simulink model "IEEE_BUS_68_Baseline"  (R2025a)
settings: Solver=ode23tb  StartTime=0.0  StopTime=150  FixedStep=Ts  MaxStep=0.0001  RelTol=1e-3
PreLoadFcn:
  | PSSMODEL=1;
  | LPSS=0;
  | WAPSS=0;
  | WAPSS2=0;
  | Ts=50e-5;
InitFcn:
  | PSSMODEL=1;
  | LPSS=0;
  | WAPSS=0;
  | WAPSS2=0;
  | Ts=50e-5;
  | 
  | % Required data to 68 Bus benchmark
  | % clear
  | % clc
  | % Definition for the columns
  | % system base =100 MVA
  | 
  | %% Line data Format (line)
  | % All values are given on the same system base MVA
  | % 1: From bus
  | % 2: To bus
  | % 3: Resistance (pu)
  | % 4: Reactance  (pu)
  | % 5: Charge     (pu)
  | % 6: Transformer Tap Amplitute
  | % 7: base MVA
  | % 8: Nomonal Voltage (KV)
  | 
  | %1   2    3        4       5       6        7      8
  | line=[...
  | 1	54	0	     0.0181	  0	      1.025     100    13.8
  | 2	58	0	     0.025	  0	      1.070     100    13.8
  | 3	62	0	     0.02	  0	      1.070     100    13.8
  | 4	19	0.0007	 0.0142	  0	      1.070     100    13.8
  | 5	20	0.0009	 0.018	  0	      1.009     100    13.8
  | 6	22	0	     0.0143	  0	      1.025     100    13.8
  | 7	23	0.0005	 0.0272	  0	      0         100    13.8
  | 8	25	0.0006	 0.0232	  0	      1.025     100    13.8
  | 9	29	0.0008	 0.0156   0	      1.025     100    13.8
  | 10	31	0	     0.026	  0	      1.04      100    13.8
  | 11	32	0	     0.013	  0	      1.04      100    13.8
  | 12	36	0	     0.0075	  0	      1.04      100    13.8
  | 13	17	0	     0.0033	  0	      1.04      100    13.8
  | 14	41	0	     0.0015	  0	      1         100    13.8
  | 15	42	0	     0.0015	  0	      1         100    13.8
  | 16	18	0	     0.003	  0	      1         100    13.8
  | 17	36	0.0005	 0.0045	  0.32	  0         100    138
  | 17	43	0.0005	 0.0276	  0	      0         100    138
  | 18	42	0.004	 0.06	  2.25    0         100    138
  | 18	49	0.0076	 0.1141	  1.16    0	        100    138
  | 18	50	0.0012	 0.0288	  2.06	  0         100    138
  | 20	19	0.0007	 0.0138	  0       1.06	    100    138
  | 19	68	0.0016	 0.0195	  0.304	  0         100    138
  | 21	22	0.0008	 0.014	  0.2565  0	        100    138
  | 21	68	0.0008	 0.0135	  0.2548  0	        100    138
  | 22	23	0.0006	 0.0096	  0.1846  0	        100    138
  | 23	24	0.0022	 0.035	  0.361	  0         100    138
  | 24	68	0.0003	 0.0059	  0.068	  0         100    138
  | 25	26	0.0032	 0.0323	  0.531	  0         100    138
  | 25	54	0.007	 0.0086	  0.146	  0         100    138
  | 26	27	0.0014	 0.0147	  0.2396  0	        100    138
  | 26	28	0.0043	 0.0474	  0.7802  0	        100    138
  | 26	29	0.0057	 0.0625	  1.029	  0         100    138
  | 27	37	0.0013	 0.0173	  0.3216  0	        100    138
  | 27	53	0.032	 0.32	  0.41	  0         100    138
  | ... (+206 lines)
undefined symbols (not defined in the file or in its folder): D1, Delta
libraries: spsRMSLib x73, spsThreePhaseVIMeasurementLib x69, spsLoadFlowBusLib x69, spsThreePhasePISectionLineLib x64, spsThreePhaseParallelRLCLoadLib x35, spsGenericPowerSystemStabilizerLib x32, spsThreePhaseSeriesRLCLoadLib x21, spsThreePhaseTransformerTwoWindingsLib x21, spsSynchronousMachinepuStandardLib x19, spsExcitationSystemLib x16, spsMultiBandPowerSystemStabilizerLib x16, spsSteamTurbineandGovernorLib x16
(part 2 of 7)

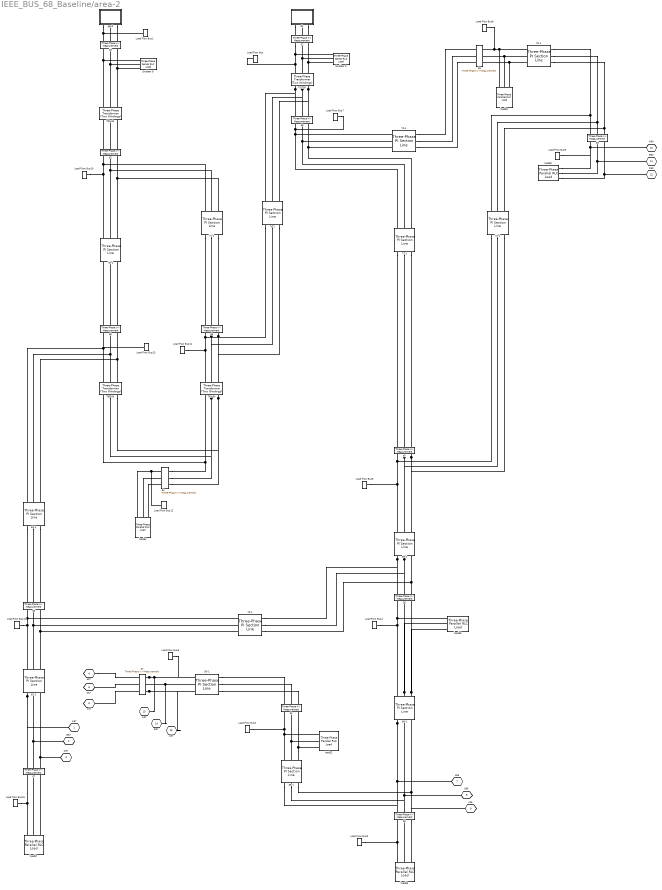
== system IEEE_BUS_68_Baseline/area-2 ==
  02 : spsThreePhaseVIMeasurementLib/Three-Phase V-I Measurement  VoltageMeasurement=phase-to-phase  SetLabelV=on  LabelV=Vabc_02  Vpu=off  VpuLL=on  CurrentMeasurement=no  SetLabelI=off  LabelI=Iabc  Ipu=off  Pbase=100e6  Vbase=13.8e3  OutputType=Complex  PhasorSimulation=off  PSBequivalent=0
  03 : spsThreePhaseVIMeasurementLib/Three-Phase V-I Measurement  VoltageMeasurement=phase-to-phase  SetLabelV=on  LabelV=Vabc_03  Vpu=off  VpuLL=on  CurrentMeasurement=no  SetLabelI=off  LabelI=Iabc  Ipu=off  Pbase=100e6  Vbase=13.8e3  OutputType=Complex  PhasorSimulation=off  PSBequivalent=0
  37 : spsThreePhaseVIMeasurementLib/Three-Phase V-I Measurement  VoltageMeasurement=phase-to-phase  SetLabelV=on  LabelV=Vabc_37  Vpu=off  VpuLL=on  CurrentMeasurement=no  SetLabelI=off  LabelI=Iabc  Ipu=off  Pbase=100e6  Vbase=Bus(37,2)*1e3  OutputType=Complex  PhasorSimulation=off  PSBequivalent=0
  50-1 : spsThreePhasePISectionLineLib/Three-Phase PI Section Line  LConnTagsString=a|b|c  RConnTagsString=A|B|C  Length=1  Frequency=60  Resistances=[line(50,3) 3*line(50,3)]  Inductances=[line(50,4) 3*line(50,4)]  Capacitances=[line(50,5) line(50,5)/3]
  52 : spsThreePhaseVIMeasurementLib/Three-Phase V-I Measurement  VoltageMeasurement=phase-to-phase  SetLabelV=on  LabelV=Vabc_52  Vpu=off  VpuLL=on  CurrentMeasurement=no  SetLabelI=off  LabelI=Iabc  Ipu=off  Pbase=100e6  Vbase=Bus(52,2)*1e3  OutputType=Complex  PhasorSimulation=off  PSBequivalent=0
  55 : spsThreePhaseVIMeasurementLib/Three-Phase V-I Measurement  VoltageMeasurement=phase-to-phase  SetLabelV=on  LabelV=Vabc_55  Vpu=off  VpuLL=on  CurrentMeasurement=no  SetLabelI=off  LabelI=Iabc  Ipu=off  Pbase=100e6  Vbase=Bus(55,2)*1e3  OutputType=Complex  PhasorSimulation=off  PSBequivalent=0
  56 : spsThreePhaseVIMeasurementLib/Three-Phase V-I Measurement  VoltageMeasurement=phase-to-phase  SetLabelV=on  LabelV=Vabc_56  Vpu=off  VpuLL=on  CurrentMeasurement=no  SetLabelI=off  LabelI=Iabc  Ipu=off  Pbase=100e6  Vbase=Bus(56,2)*1e3  OutputType=Complex  PhasorSimulation=off  PSBequivalent=0
  57 : spsThreePhaseVIMeasurementLib/Three-Phase V-I Measurement  VoltageMeasurement=phase-to-phase  SetLabelV=on  LabelV=Vabc_57  Vpu=off  VpuLL=on  CurrentMeasurement=no  SetLabelI=off  LabelI=Iabc  Ipu=off  Pbase=100e6  Vbase=Bus(57,2)*1e3  OutputType=Complex  PhasorSimulation=off  PSBequivalent=0
  58 : spsThreePhaseVIMeasurementLib/Three-Phase V-I Measurement  VoltageMeasurement=phase-to-phase  SetLabelV=on  LabelV=Vabc_58  Vpu=off  VpuLL=on  CurrentMeasurement=no  SetLabelI=off  LabelI=Iabc  Ipu=off  Pbase=100e6  Vbase=Bus(58,2)*1e3  OutputType=Complex  PhasorSimulation=off  PSBequivalent=0
  59 : spsThreePhaseVIMeasurementLib/Three-Phase V-I Measurement  VoltageMeasurement=phase-to-phase  SetLabelV=on  LabelV=Vabc_59  Vpu=off  VpuLL=on  CurrentMeasurement=no  SetLabelI=off  LabelI=Iabc  Ipu=off  Pbase=100e6  Vbase=Bus(59,2)*1e3  OutputType=Complex  PhasorSimulation=off  PSBequivalent=0
  60 : spsThreePhaseVIMeasurementLib/Three-Phase V-I Measurement  VoltageMeasurement=phase-to-phase  SetLabelV=on  LabelV=Vabc_60  Vpu=off  VpuLL=on  CurrentMeasurement=no  SetLabelI=off  LabelI=Iabc  Ipu=off  Pbase=100e6  Vbase=Bus(60,2)*1e3  OutputType=Complex  PhasorSimulation=off  PSBequivalent=0
  62 : spsThreePhaseVIMeasurementLib/Three-Phase V-I Measurement  VoltageMeasurement=phase-to-phase  SetLabelV=on  LabelV=Vabc_62  Vpu=off  VpuLL=on  CurrentMeasurement=no  SetLabelI=off  LabelI=Iabc  Ipu=off  Pbase=100e6  Vbase=Bus(62,2)*1e3  OutputType=Complex  PhasorSimulation=off  PSBequivalent=0
  63 : spsThreePhaseVIMeasurementLib/Three-Phase V-I Measurement  VoltageMeasurement=phase-to-phase  SetLabelV=on  LabelV=Vabc_63  Vpu=off  VpuLL=on  CurrentMeasurement=no  SetLabelI=off  LabelI=Iabc  Ipu=off  Pbase=100e6  Vbase=Bus(63,2)*1e3  OutputType=Complex  PhasorSimulation=off  PSBequivalent=0
  64 : spsThreePhaseVIMeasurementLib/Three-Phase V-I Measurement  VoltageMeasurement=phase-to-phase  SetLabelV=on  LabelV=Vabc_64  Vpu=off  VpuLL=on  CurrentMeasurement=no  SetLabelI=off  LabelI=Iabc  Ipu=off  Pbase=100e6  Vbase=Bus(64,2)*1e3  OutputType=Complex  PhasorSimulation=off  PSBequivalent=0
  65 : spsThreePhaseVIMeasurementLib/Three-Phase V-I Measurement  VoltageMeasurement=phase-to-phase  SetLabelV=on  LabelV=Vabc_65  Vpu=off  VpuLL=on  CurrentMeasurement=no  SetLabelI=off  LabelI=Iabc  Ipu=off  Pbase=100e6  Vbase=Bus(65,2)*1e3  OutputType=Complex  PhasorSimulation=off  PSBequivalent=0
  65-1 : spsThreePhasePISectionLineLib/Three-Phase PI Section Line  LConnTagsString=a|b|c  RConnTagsString=A|B|C  Length=1  Frequency=60  Resistances=[line(65,3) 3*line(65,3)]  Inductances=[line(65,4) 3*line(65,4)]  Capacitances=[line(65,5) line(65,5)/3]
  66 : spsThreePhaseVIMeasurementLib/Three-Phase V-I Measurement  VoltageMeasurement=phase-to-phase  SetLabelV=on  LabelV=Vabc_66  Vpu=off  VpuLL=on  CurrentMeasurement=no  SetLabelI=off  LabelI=Iabc  Ipu=off  Pbase=100e6  Vbase=Bus(66,2)*1e3  OutputType=Complex  PhasorSimulation=off  PSBequivalent=0
  67 : spsThreePhaseVIMeasurementLib/Three-Phase V-I Measurement  VoltageMeasurement=phase-to-phase  SetLabelV=on  LabelV=Vabc_67  Vpu=off  VpuLL=on  CurrentMeasurement=no  SetLabelI=off  LabelI=Iabc  Ipu=off  Pbase=100e6  Vbase=Bus(67,2)*1e3  OutputType=Complex  PhasorSimulation=off  PSBequivalent=0
  68-1 : spsThreePhasePISectionLineLib/Three-Phase PI Section Line  LConnTagsString=a|b|c  RConnTagsString=A|B|C  Length=1  Frequency=60  Resistances=[line(68,3) 3*line(68,3)]  Inductances=[line(68,4) 3*line(68,4)]  Capacitances=[line(68,5) line(68,5)/3]
  69-1 : spsThreePhasePISectionLineLib/Three-Phase PI Section Line  LConnTagsString=a|b|c  RConnTagsString=A|B|C  Length=1  Frequency=60  Resistances=[line(69,3) 3*line(69,3)]  Inductances=[line(69,4) 3*line(69,4)]  Capacitances=[line(69,5) line(69,5)/3]
  70-1 : spsThreePhasePISectionLineLib/Three-Phase PI Section Line  LConnTagsString=a|b|c  RConnTagsString=A|B|C  Length=1  Frequency=60  Resistances=[line(70,3) 3*line(70,3)]  Inductances=[line(70,4) 3*line(70,4)]  Capacitances=[line(70,5) line(70,5)/3]
  71-1 : spsThreePhasePISectionLineLib/Three-Phase PI Section Line  LConnTagsString=a|b|c  RConnTagsString=A|B|C  Length=1  Frequency=60  Resistances=[line(71,3) 3*line(71,3)]  Inductances=[line(71,4) 3*line(71,4)]  Capacitances=[line(71,5) line(71,5)/3]
  72-1 : spsThreePhasePISectionLineLib/Three-Phase PI Section Line  LConnTagsString=a|b|c  RConnTagsString=A|B|C  Length=1  Frequency=60  Resistances=[line(72,3) 3*line(72,3)]  Inductances=[line(72,4) 3*line(72,4)]  Capacitances=[line(72,5) line(72,5)/3]
  73-1 : spsThreePhasePISectionLineLib/Three-Phase PI Section Line  LConnTagsString=a|b|c  RConnTagsString=A|B|C  Length=1  Frequency=60  Resistances=[line(73,3) 3*line(73,3)]  Inductances=[line(73,4) 3*line(73,4)]  Capacitances=[line(73,5) line(73,5)/3]
  74-1 : spsThreePhasePISectionLineLib/Three-Phase PI Section Line  LConnTagsString=a|b|c  RConnTagsString=A|B|C  Length=1  Frequency=60  Resistances=[line(74,3) 3*line(74,3)]  Inductances=[line(74,4) 3*line(74,4)]  Capacitances=[line(74,5) line(74,5)/3]
  75-1 : spsThreePhasePISectionLineLib/Three-Phase PI Section Line  LConnTagsString=a|b|c  RConnTagsString=A|B|C  Length=1  Frequency=60  Resistances=[line(75,3) 3*line(75,3)]  Inductances=[line(75,4) 3*line(75,4)]  Capacitances=[line(75,5) line(75,5)/3]
  77-1 : spsThreePhasePISectionLineLib/Three-Phase PI Section Line  LConnTagsString=a|b|c  RConnTagsString=A|B|C  Length=1  Frequency=60  Resistances=[line(77,3) 3*line(77,3)]  Inductances=[line(77,4) 3*line(77,4)]  Capacitances=[line(77,5) line(77,5)/3]
  78-1 : spsThreePhasePISectionLineLib/Three-Phase PI Section Line  LConnTagsString=a|b|c  RConnTagsString=A|B|C  Length=1  Frequency=60  Resistances=[line(78,3) 3*line(78,3)]  Inductances=[line(78,4) 3*line(78,4)]  Capacitances=[line(78,5) line(78,5)/3]
  81-1 : spsThreePhasePISectionLineLib/Three-Phase PI Section Line  LConnTagsString=a|b|c  RConnTagsString=A|B|C  Length=1  Frequency=60  Resistances=[line(81,3) 3*line(81,3)]  Inductances=[line(81,4) 3*line(81,4)]  Capacitances=[line(81,5) line(81,5)/3]
  81-2 : spsThreePhasePISectionLineLib/Three-Phase PI Section Line  LConnTagsString=a|b|c  RConnTagsString=A|B|C  Length=1  Frequency=60  Resistances=[line(81,3) 3*line(81,3)]  Inductances=[line(81,4) 3*line(81,4)]  Capacitances=[line(81,5) line(81,5)/3]
  G2 : Subsystem
  Load Flow Bus : spsLoadFlowBusLib/Load Flow Bus  LConnTagsString=a  Phases=single  Connectors=on one side  ID=BUS_02  Vbase=13.8e3  Vref=0.98  Vangle=0  VLF=0.98  VLFb=1  VLFc=1  angleLF=-3.815  angleLFb=0  angleLFc=0
  Load Flow Bus1 : spsLoadFlowBusLib/Load Flow Bus  LConnTagsString=a  Phases=single  Connectors=on one side  ID=BUS_03  Vbase=13.8e3  Vref=0.983  Vangle=0  VLF=0.983  VLFb=1  VLFc=1  angleLF=2.903  angleLFb=0  angleLFc=0
  Load Flow Bus10 : spsLoadFlowBusLib/Load Flow Bus  LConnTagsString=a  Phases=single  Connectors=on one side  ID=BUS_62  Vbase=138e3  Vref=1  Vangle=0  VLF=0.9822  VLFb=1  VLFc=1  angleLF=29.01  angleLFb=0  angleLFc=0
  Load Flow Bus11 : spsLoadFlowBusLib/Load Flow Bus  LConnTagsString=a  Phases=single  Connectors=on one side  ID=BUS_63  Vbase=138e3  Vref=1  Vangle=0  VLF=0.9798  VLFb=1  VLFc=1  angleLF=28.04  angleLFb=0  angleLFc=0
  Load Flow Bus12 : spsLoadFlowBusLib/Load Flow Bus  LConnTagsString=a  Phases=single  Connectors=on one side  ID=BUS_64  Vbase=138e3  Vref=1  Vangle=0  VLF=0.971  VLFb=1  VLFc=1  angleLF=28.2  angleLFb=0  angleLFc=0
  Load Flow Bus13 : spsLoadFlowBusLib/Load Flow Bus  LConnTagsString=a  Phases=single  Connectors=on one side  ID=BUS_65  Vbase=138e3  Vref=1  Vangle=0  VLF=0.9825  VLFb=1  VLFc=1  angleLF=28.32  angleLFb=0  angleLFc=0
  Load Flow Bus14 : spsLoadFlowBusLib/Load Flow Bus  LConnTagsString=a  Phases=single  Connectors=on one side  ID=BUS_66  Vbase=138e3  Vref=1  Vangle=0  VLF=0.9879  VLFb=1  VLFc=1  angleLF=26.8  angleLFb=0  angleLFc=0
  Load Flow Bus15 : spsLoadFlowBusLib/Load Flow Bus  LConnTagsString=a  Phases=single  Connectors=on one side  ID=BUS_67  Vbase=138e3  Vref=1  Vangle=0  VLF=0.9975  VLFb=1  VLFc=1  angleLF=26.93  angleLFb=0  angleLFc=0
  Load Flow Bus2 : spsLoadFlowBusLib/Load Flow Bus  LConnTagsString=a  Phases=single  Connectors=on one side  ID=BUS_52  Vbase=138e3  Vref=1  Vangle=0  VLF=1.004  VLFb=1  VLFc=1  angleLF=24.49  angleLFb=0  angleLFc=0
  Load Flow Bus3 : spsLoadFlowBusLib/Load Flow Bus  LConnTagsString=a  Phases=single  Connectors=on one side  ID=BUS_55  Vbase=138e3  Vref=1  Vangle=0  VLF=0.9927  VLFb=1  VLFc=1  angleLF=22.46  angleLFb=0  angleLFc=0
  Load Flow Bus4 : spsLoadFlowBusLib/Load Flow Bus  LConnTagsString=a  Phases=single  Connectors=on one side  ID=BUS_56  Vbase=138e3  Vref=1  Vangle=0  VLF=0.9814  VLFb=1  VLFc=1  angleLF=24.68  angleLFb=0  angleLFc=0
  Load Flow Bus5 : spsLoadFlowBusLib/Load Flow Bus  LConnTagsString=a  Phases=single  Connectors=on one side  ID=BUS_37  Vbase=138e3  Vref=1  Vangle=0  VLF=1.011  VLFb=1  VLFc=1  angleLF=25.73  angleLFb=0  angleLFc=0
  Load Flow Bus6 : spsLoadFlowBusLib/Load Flow Bus  LConnTagsString=a  Phases=single  Connectors=on one side  ID=BUS_57  Vbase=138e3  Vref=1  Vangle=0  VLF=0.9776  VLFb=1  VLFc=1  angleLF=25.41  angleLFb=0  angleLFc=0
  Load Flow Bus7 : spsLoadFlowBusLib/Load Flow Bus  LConnTagsString=a  Phases=single  Connectors=on one side  ID=BUS_58  Vbase=138e3  Vref=1  Vangle=0  VLF=0.9787  VLFb=1  VLFc=1  angleLF=26.13  angleLFb=0  angleLFc=0
  Load Flow Bus8 : spsLoadFlowBusLib/Load Flow Bus  LConnTagsString=a  Phases=single  Connectors=on one side  ID=BUS_59  Vbase=138e3  Vref=1  Vangle=0  VLF=0.9693  VLFb=1  VLFc=1  angleLF=23.58  angleLFb=0  angleLFc=0
  Load Flow Bus9 : spsLoadFlowBusLib/Load Flow Bus  LConnTagsString=a  Phases=single  Connectors=on one side  ID=BUS_60  Vbase=138e3  Vref=1  Vangle=0  VLF=0.9693  VLFb=1  VLFc=1  angleLF=22.93  angleLFb=0  angleLFc=0
  Snubber 8 : spsThreePhaseSeriesRLCLoadLib/Three-Phase Series RLC Load  LConnTagsString=A|B|C  Configuration=Y (grounded)  NominalVoltage=13.8e3  Vabc=[1e3 1e3 1e3]  Vabcp=[1e3 1e3 1e3]  NominalFrequency=60  UnbalancedPower=off  ActivePower=1000000  InductivePower=0  CapacitivePower=10000000  Pabc=[10e3 9e3 11e3]  QLabc=[100 90 110]  QCabc=[100 90 110]  Pabcp=[10e3 9e3 11e3]  QLabcp=[100 90 110]  QCabcp=[100 90 110]  Measurements=None  LoadType=constant Z
  Snubber 9 : spsThreePhaseSeriesRLCLoadLib/Three-Phase Series RLC Load  LConnTagsString=A|B|C  Configuration=Y (grounded)  NominalVoltage=13.8e3  Vabc=[1e3 1e3 1e3]  Vabcp=[1e3 1e3 1e3]  NominalFrequency=60  UnbalancedPower=off  ActivePower=1000000  InductivePower=0  CapacitivePower=10000000  Pabc=[10e3 9e3 11e3]  QLabc=[100 90 110]  QCabc=[100 90 110]  Pabcp=[10e3 9e3 11e3]  QLabcp=[100 90 110]  QCabcp=[100 90 110]  Measurements=None  LoadType=constant Z
  T02-58 : spsThreePhaseTransformerTwoWindingsLib/Three-Phase Transformer (Two Windings)  Winding1Connection=Delta (D1)  Winding2Connection=Yg  CoreType=Three single-phase transformers  SetSaturation=off  Hysteresis=off  DataFile='hysteresis'  SetInitialFlux=off  Measurements=None  UNITS=pu  NominalPower=[ 100e6 , 60 ]  Winding1=[ 13.8e3 , 0.0002 , 0 ]  Winding2=[ 138e3 , 0 .0002, 0.0125]  Rm=500  Lm=500  L0=0.5  Saturation=[ 0,0 ; 0.0024,1.2 ; 1.0,1.52 ]  InitialFluxes=[ 0.8 , -0.8 , 0.7 ]  BreakLoop=off  DiscreteSolver=Trapezoidal robust  DataType=off  TransfoNumber=1
  T03-62 : spsThreePhaseTransformerTwoWindingsLib/Three-Phase Transformer (Two Windings)  Winding1Connection=Delta (D1)  Winding2Connection=Yg  CoreType=Three single-phase transformers  SetSaturation=off  Hysteresis=off  DataFile='hysteresis'  SetInitialFlux=off  Measurements=None  UNITS=pu  NominalPower=[ 100e6 , 60 ]  Winding1=[ 13.8e3 , 0.000 , 0 ]  Winding2=[ 138e3 , 0.000, 0.0101]  Rm=500  Lm=500  L0=0.5  Saturation=[ 0,0 ; 0.0024,1.2 ; 1.0,1.52 ]  InitialFluxes=[ 0.8 , -0.8 , 0.7 ]  BreakLoop=off  DiscreteSolver=Trapezoidal robust  DataType=off  TransfoNumber=1
  T63-64 : spsThreePhaseTransformerTwoWindingsLib/Three-Phase Transformer (Two Windings)  Winding1Connection=Y  Winding2Connection=Y  CoreType=Three single-phase transformers  SetSaturation=off  Hysteresis=off  DataFile='hysteresis'  SetInitialFlux=off  Measurements=None  UNITS=pu  NominalPower=[ 100e6 , 60 ]  Winding1=[ 138e3 , 0.00152, 0 ]  Winding2=[ 138e3 , 0.00152 , 0.022]  Rm=500  Lm=500  L0=0.5  Saturation=[ 0,0 ; 0.0024,1.2 ; 1.0,1.52 ]  InitialFluxes=[ 0.8 , -0.8 , 0.7 ]  BreakLoop=off  DiscreteSolver=Trapezoidal robust  DataType=off  TransfoNumber=1
  T65-64 : spsThreePhaseTransformerTwoWindingsLib/Three-Phase Transformer (Two Windings)  Winding1Connection=Y  Winding2Connection=Y  CoreType=Three single-phase transformers  SetSaturation=off  Hysteresis=off  DataFile='hysteresis'  SetInitialFlux=off  Measurements=None  UNITS=pu  NominalPower=[ 100e6 , 60 ]  Winding1=[ 138e3 , 0.00152, 0 ]  Winding2=[ 138e3 , 0.00152 , 0.022]  Rm=500  Lm=500  L0=0.5  Saturation=[ 0,0 ; 0.0024,1.2 ; 1.0,1.52 ]  InitialFluxes=[ 0.8 , -0.8 , 0.7 ]  BreakLoop=off  DiscreteSolver=Trapezoidal robust  DataType=off  TransfoNumber=1
  gen3 : Subsystem
  load52 : spsThreePhaseParallelRLCLoadLib/Three-Phase Parallel RLC Load  LConnTagsString=A|B|C  Configuration=Y (grounded)  NominalVoltage=(138000)*1.00427  Vabc=[1e3 1e3 1e3]  Vabcp=[1e3 1e3 1e3]  NominalFrequency=60  UnbalancedPower=off  ActivePower=2000000  InductivePower=460000  CapacitivePower=0  Pabc=[10e3 9e3 11e3]  QLabc=[100 90 110]  QCabc=[100 90 110]  Pabcp=[10e3 9e3 11e3]  QLabcp=[100 90 110]  QCabcp=[100 90 110]  Measurements=None  LoadType=constant PQ
  load55 : spsThreePhaseParallelRLCLoadLib/Three-Phase Parallel RLC Load  LConnTagsString=A|B|C  Configuration=Y (grounded)  NominalVoltage=(138000)*0.992749  Vabc=[1e3 1e3 1e3]  Vabcp=[1e3 1e3 1e3]  NominalFrequency=60  UnbalancedPower=off  ActivePower=680000000  InductivePower=157000000  CapacitivePower=0  Pabc=[10e3 9e3 11e3]  QLabc=[100 90 110]  QCabc=[100 90 110]  Pabcp=[10e3 9e3 11e3]  QLabcp=[100 90 110]  QCabcp=[100 90 110]  Measurements=None  LoadType=constant PQ
  load56 : spsThreePhaseParallelRLCLoadLib/Three-Phase Parallel RLC Load  LConnTagsString=A|B|C  Configuration=Y (grounded)  NominalVoltage=(138000)*0.981401  Vabc=[1e3 1e3 1e3]  Vabcp=[1e3 1e3 1e3]  NominalFrequency=60  UnbalancedPower=off  ActivePower=200000000  InductivePower=74000000  CapacitivePower=0  Pabc=[10e3 9e3 11e3]  QLabc=[100 90 110]  QCabc=[100 90 110]  Pabcp=[10e3 9e3 11e3]  QLabcp=[100 90 110]  QCabcp=[100 90 110]  Measurements=None  LoadType=constant PQ
  load59 : spsThreePhaseParallelRLCLoadLib/Three-Phase Parallel RLC Load  LConnTagsString=A|B|C  Configuration=Y (grounded)  NominalVoltage=(138000)*0.969335  Vabc=[1e3 1e3 1e3]  Vabcp=[1e3 1e3 1e3]  NominalFrequency=60  UnbalancedPower=off  ActivePower=234000000  InductivePower=84000000  CapacitivePower=0  Pabc=[10e3 9e3 11e3]  QLabc=[100 90 110]  QCabc=[100 90 110]  Pabcp=[10e3 9e3 11e3]  QLabcp=[100 90 110]  QCabcp=[100 90 110]  Measurements=None  LoadType=constant PQ
  load60 : spsThreePhaseParallelRLCLoadLib/Three-Phase Parallel RLC Load  LConnTagsString=A|B|C  Configuration=Y (grounded)  NominalVoltage=(138000)*0.969257  Vabc=[1e3 1e3 1e3]  Vabcp=[1e3 1e3 1e3]  NominalFrequency=60  UnbalancedPower=off  ActivePower=209000000  InductivePower=71000000  CapacitivePower=0  Pabc=[10e3 9e3 11e3]  QLabc=[100 90 110]  QCabc=[100 90 110]  Pabcp=[10e3 9e3 11e3]  QLabcp=[100 90 110]  QCabcp=[100 90 110]  Measurements=None  LoadType=constant PQ
  load64 : spsThreePhaseParallelRLCLoadLib/Three-Phase Parallel RLC Load  LConnTagsString=A|B|C  Configuration=Y (grounded)  NominalVoltage=(138000)*0.971036  Vabc=[1e3 1e3 1e3]  Vabcp=[1e3 1e3 1e3]  NominalFrequency=60  UnbalancedPower=off  ActivePower=9000000  InductivePower=88000000  CapacitivePower=0  Pabc=[10e3 9e3 11e3]  QLabc=[100 90 110]  QCabc=[100 90 110]  Pabcp=[10e3 9e3 11e3]  QLabcp=[100 90 110]  QCabcp=[100 90 110]  Measurements=None  LoadType=constant PQ
  load67 : spsThreePhaseParallelRLCLoadLib/Three-Phase Parallel RLC Load  LConnTagsString=A|B|C  Configuration=Y (grounded)  NominalVoltage=(138000)*0.997526  Vabc=[1e3 1e3 1e3]  Vabcp=[1e3 1e3 1e3]  NominalFrequency=60  UnbalancedPower=off  ActivePower=118000000  InductivePower=27000000  CapacitivePower=0  Pabc=[10e3 9e3 11e3]  QLabc=[100 90 110]  QCabc=[100 90 110]  Pabcp=[10e3 9e3 11e3]  QLabcp=[100 90 110]  QCabcp=[100 90 110]  Measurements=None  LoadType=constant PQ
  A67 : PMIOPort  Tag=PMCPort  Side=Right
  B67 : PMIOPort  Tag=PMCPort  Port=2  Side=Right
  C67 : PMIOPort  Tag=PMCPort  Port=3  Side=Right
  a37 : PMIOPort  Tag=PMCPort  Port=4  Side=Right
  c37 : PMIOPort  Tag=PMCPort  Port=5  Side=Right
  b37 : PMIOPort  Tag=PMCPort  Port=6  Side=Right
  a55 : PMIOPort  Tag=PMCPort  Port=7  Side=Right
  b55 : PMIOPort  Tag=PMCPort  Port=8  Side=Right
  c55 : PMIOPort  Tag=PMCPort  Port=9  Side=Right
  A60 : PMIOPort  Tag=PMCPort  Port=10  Side=Right
  B60 : PMIOPort  Tag=PMCPort  Port=11  Side=Right
  C60 : PMIOPort  Tag=PMCPort  Port=12  Side=Right
  A37 : PMIOPort  Tag=PMCPort  Port=13  Side=Right
  B37 : PMIOPort  Tag=PMCPort  Port=14  Side=Right
  C37 : PMIOPort  Tag=PMCPort  Port=15  Side=Right
  connections:
  gen3/LConn2 -- 03/RConn2
  62/RConn3 -- T03-62/RConn3
  T03-62/LConn1 -- 03/LConn1 -- Snubber 8/LConn1
  T03-62/LConn2 -- 03/LConn2 -- Snubber 8/LConn2
  62/RConn2 -- T03-62/RConn2
  62/RConn1 -- T03-62/RConn1
  gen3/LConn3 -- 03/RConn3
  gen3/LConn1 -- Load Flow Bus1/LConn1 -- 03/RConn1
  T03-62/LConn3 -- Snubber 8/LConn3 -- 03/LConn3
  78-1/RConn1 -- Load Flow Bus10/LConn1 -- 77-1/RConn1 -- 62/LConn1
  78-1/RConn2 -- 77-1/RConn2 -- 62/LConn2
  78-1/RConn3 -- 77-1/RConn3 -- 62/LConn3
  65/RConn1 -- 78-1/LConn1
  65/RConn2 -- 78-1/LConn2
  65/RConn3 -- 78-1/LConn3
  77-1/LConn1 -- 63/RConn1
  77-1/LConn2 -- 63/RConn2
  77-1/LConn3 -- 63/RConn3
  T63-64/LConn1 -- Load Flow Bus11/LConn1 -- 63/LConn1 -- 74-1/RConn1
  63/LConn2 -- T63-64/LConn2 -- 74-1/RConn2
  63/LConn3 -- T63-64/LConn3 -- 74-1/RConn3
  64/RConn1 -- T63-64/RConn1 -- T65-64/RConn1
  T63-64/RConn2 -- 64/RConn2 -- T65-64/RConn2
  T63-64/RConn3 -- 64/RConn3 -- T65-64/RConn3
  T65-64/LConn1 -- Load Flow Bus13/LConn1 -- 65/LConn1 -- 81-1/RConn1
  T65-64/LConn2 -- 81-1/RConn2 -- 65/LConn2
  T65-64/LConn3 -- 81-1/RConn3 -- 65/LConn3
  load64/LConn1 -- Load Flow Bus12/LConn1 -- 64/LConn1
  load64/LConn2 -- 64/LConn2
  load64/LConn3 -- 64/LConn3
  81-1/LConn1 -- 66/RConn1
  81-1/LConn2 -- 66/RConn2
  81-1/LConn3 -- 66/RConn3
  81-2/RConn1 -- Load Flow Bus14/LConn1 -- 66/LConn1 -- 70-1/RConn1
  81-2/RConn2 -- 66/LConn2 -- 70-1/RConn2
  81-2/RConn3 -- 66/LConn3 -- 70-1/RConn3
  81-2/LConn1 -- 67/RConn1 -- A67/RConn1
  67/RConn2 -- 81-2/LConn2 -- B67/RConn1
  C67/RConn1 -- 67/RConn3 -- 81-2/LConn3
  G2/LConn1 -- 02/RConn1
  G2/LConn2 -- 02/RConn2
  G2/LConn3 -- 02/RConn3
  02/LConn1 -- Snubber 9/LConn1 -- Load Flow Bus/LConn1 -- T02-58/LConn1
  T02-58/LConn2 -- 02/LConn2 -- Snubber 9/LConn2
  T02-58/LConn3 -- Snubber 9/LConn3 -- 02/LConn3
  T02-58/RConn1 -- 58/RConn1 -- 74-1/LConn1
  T02-58/RConn2 -- 58/RConn2 -- 74-1/LConn2
  T02-58/RConn3 -- 58/RConn3 -- 74-1/LConn3
  73-1/RConn1 -- 71-1/RConn1 -- Load Flow Bus7/LConn1 -- 58/LConn1
  71-1/RConn2 -- 73-1/RConn2 -- 58/LConn2
  71-1/RConn3 -- 73-1/RConn3 -- 58/LConn3
  71-1/LConn1 -- 57/RConn1
  71-1/LConn2 -- 57/RConn2
  71-1/LConn3 -- 57/RConn3
  73-1/LConn1 -- 59/RConn1
  73-1/LConn2 -- 59/RConn2
  73-1/LConn3 -- 59/RConn3
  75-1/RConn1 -- load59/LConn1 -- Load Flow Bus8/LConn1 -- 59/LConn1
  75-1/RConn2 -- load59/LConn2 -- 59/LConn2
  75-1/RConn3 -- load59/LConn3 -- 59/LConn3
  75-1/LConn1 -- 60/RConn1 -- 72-1/LConn1
  75-1/LConn2 -- 60/RConn2 -- 72-1/LConn2
  75-1/LConn3 -- 60/RConn3 -- 72-1/LConn3
  A60/RConn1 -- load60/LConn1 -- Load Flow Bus9/LConn1 -- 60/LConn1
  load60/LConn2 -- 60/LConn2 -- B60/RConn1
  load60/LConn3 -- C60/RConn1 -- 60/LConn3
  69-1/RConn1 -- 57/LConn1 -- 72-1/RConn1 -- Load Flow Bus6/LConn1
  57/LConn2 -- 69-1/RConn2 -- 72-1/RConn2
  57/LConn3 -- 69-1/RConn3 -- 72-1/RConn3
  69-1/LConn1 -- 56/RConn1 -- 70-1/LConn1
  69-1/LConn2 -- 56/RConn2 -- 70-1/LConn2
  56/RConn3 -- 70-1/LConn3 -- 69-1/LConn3
  68-1/RConn1 -- Load Flow Bus4/LConn1 -- load56/LConn1 -- 56/LConn1
  68-1/RConn2 -- load56/LConn2 -- 56/LConn2
  68-1/RConn3 -- load56/LConn3 -- 56/LConn3
  68-1/LConn1 -- 55/RConn1 -- 65-1/LConn1 -- a55/RConn1
  b55/RConn1 -- 55/RConn2 -- 65-1/LConn2 -- 68-1/LConn2
  65-1/LConn3 -- 68-1/LConn3 -- 55/RConn3 -- c55/RConn1
  load67/LConn1 -- Load Flow Bus15/LConn1 -- 67/LConn1
  load67/LConn2 -- 67/LConn2
  load67/LConn3 -- 67/LConn3
  65-1/RConn1 -- 52/LConn1 -- Load Flow Bus2/LConn1 -- load52/LConn1
  65-1/RConn2 -- load52/LConn2 -- 52/LConn2
  65-1/RConn3 -- load52/LConn3 -- 52/LConn3
  Load Flow Bus3/LConn1 -- 55/LConn1 -- load55/LConn1
  a37/RConn1 -- 37/RConn1
  37/RConn2 -- b37/RConn1
  37/RConn3 -- c37/RConn1
  37/LConn1 -- Load Flow Bus5/LConn1 -- 50-1/RConn1 -- A37/RConn1
  50-1/RConn2 -- B37/RConn1 -- 37/LConn2
  37/LConn3 -- 50-1/RConn3 -- C37/RConn1
  50-1/LConn1 -- 52/RConn1
  50-1/LConn2 -- 52/RConn2
  50-1/LConn3 -- 52/RConn3
  load55/LConn2 -- 55/LConn2
  load55/LConn3 -- 55/LConn3

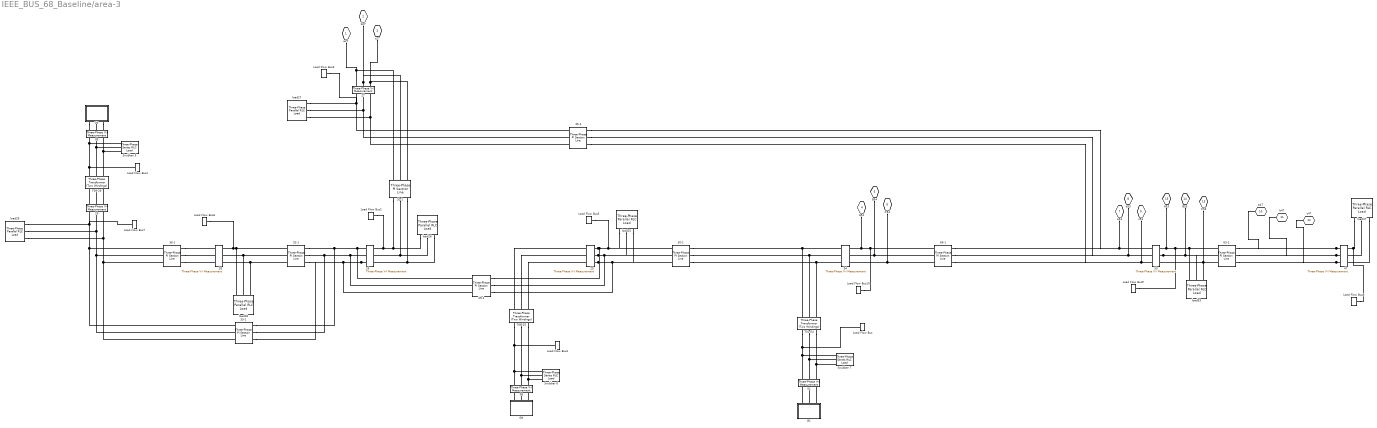
== system IEEE_BUS_68_Baseline/area-3 ==
  01 : spsThreePhaseVIMeasurementLib/Three-Phase V-I Measurement  VoltageMeasurement=phase-to-phase  SetLabelV=on  LabelV=Vabc_01  Vpu=off  VpuLL=on  CurrentMeasurement=no  SetLabelI=off  LabelI=Iabc  Ipu=off  Pbase=100e6  Vbase=13.8e3  OutputType=Complex  PhasorSimulation=off  PSBequivalent=0
  08 : spsThreePhaseVIMeasurementLib/Three-Phase V-I Measurement  VoltageMeasurement=phase-to-phase  SetLabelV=on  LabelV=Vabc_08  Vpu=off  VpuLL=on  CurrentMeasurement=no  SetLabelI=off  LabelI=Iabc  Ipu=off  Pbase=100e6  Vbase=13.8e3  OutputType=Complex  PhasorSimulation=off  PSBequivalent=0
  09 : spsThreePhaseVIMeasurementLib/Three-Phase V-I Measurement  VoltageMeasurement=phase-to-phase  SetLabelV=on  LabelV=Vabc_09  Vpu=off  VpuLL=on  CurrentMeasurement=no  SetLabelI=off  LabelI=Iabc  Ipu=off  Pbase=100e6  Vbase=13.8e3  OutputType=Complex  PhasorSimulation=off  PSBequivalent=0
  25 : spsThreePhaseVIMeasurementLib/Three-Phase V-I Measurement  VoltageMeasurement=phase-to-phase  SetLabelV=on  LabelV=Vabc_25  Vpu=off  VpuLL=on  CurrentMeasurement=no  SetLabelI=off  LabelI=Iabc  Ipu=off  Pbase=100e6  Vbase=Bus(25,2)*1e3  OutputType=Complex  PhasorSimulation=off  PSBequivalent=0
  26 : spsThreePhaseVIMeasurementLib/Three-Phase V-I Measurement  VoltageMeasurement=phase-to-phase  SetLabelV=on  LabelV=Vabc_26  Vpu=off  VpuLL=on  CurrentMeasurement=no  SetLabelI=off  LabelI=Iabc  Ipu=off  Pbase=100e6  Vbase=Bus(26,2)*1e3  OutputType=Complex  PhasorSimulation=off  PSBequivalent=0
  27 : spsThreePhaseVIMeasurementLib/Three-Phase V-I Measurement  VoltageMeasurement=phase-to-phase  SetLabelV=on  LabelV=Vabc_27  Vpu=off  VpuLL=on  CurrentMeasurement=no  SetLabelI=off  LabelI=Iabc  Ipu=off  Pbase=100e6  Vbase=Bus(27,2)*1e3  OutputType=Complex  PhasorSimulation=off  PSBequivalent=0
  28 : spsThreePhaseVIMeasurementLib/Three-Phase V-I Measurement  VoltageMeasurement=phase-to-phase  SetLabelV=on  LabelV=Vabc_28  Vpu=off  VpuLL=on  CurrentMeasurement=no  SetLabelI=off  LabelI=Iabc  Ipu=off  Pbase=100e6  Vbase=Bus(28,2)*1e3  OutputType=Complex  PhasorSimulation=off  PSBequivalent=0
  29 : spsThreePhaseVIMeasurementLib/Three-Phase V-I Measurement  VoltageMeasurement=phase-to-phase  SetLabelV=on  LabelV=Vabc_29  Vpu=off  VpuLL=on  CurrentMeasurement=no  SetLabelI=off  LabelI=Iabc  Ipu=off  Pbase=100e6  Vbase=Bus(29,2)*1e3  OutputType=Complex  PhasorSimulation=off  PSBequivalent=0
  29-1 : spsThreePhasePISectionLineLib/Three-Phase PI Section Line  LConnTagsString=a|b|c  RConnTagsString=A|B|C  Length=1  Frequency=60  Resistances=[line(29,3) 3*line(29,3)]  Inductances=[line(29,4) 3*line(29,4)]  Capacitances=[line(29,5) line(29,5)/3]
  30-1 : spsThreePhasePISectionLineLib/Three-Phase PI Section Line  LConnTagsString=a|b|c  RConnTagsString=A|B|C  Length=1  Frequency=60  Resistances=[line(30,3) 3*line(30,3)]  Inductances=[line(30,4) 3*line(30,4)]  Capacitances=[line(30,5) line(30,5)/3]
  31-1 : spsThreePhasePISectionLineLib/Three-Phase PI Section Line  LConnTagsString=a|b|c  RConnTagsString=A|B|C  Length=1  Frequency=60  Resistances=[line(31,3) 3*line(31,3)]  Inductances=[line(31,4) 3*line(31,4)]  Capacitances=[line(31,5) line(31,5)/3]
  32-1 : spsThreePhasePISectionLineLib/Three-Phase PI Section Line  LConnTagsString=a|b|c  RConnTagsString=A|B|C  Length=1  Frequency=60  Resistances=[line(32,3) 3*line(32,3)]  Inductances=[line(32,4) 3*line(32,4)]  Capacitances=[line(32,5) line(32,5)/3]
  33-1 : spsThreePhasePISectionLineLib/Three-Phase PI Section Line  LConnTagsString=a|b|c  RConnTagsString=A|B|C  Length=1  Frequency=60  Resistances=[line(33,3) 3*line(33,3)]  Inductances=[line(33,4) 3*line(33,4)]  Capacitances=[line(33,5) line(33,5)/3]
  35-1 : spsThreePhasePISectionLineLib/Three-Phase PI Section Line  LConnTagsString=a|b|c  RConnTagsString=A|B|C  Length=1  Frequency=60  Resistances=[line(35,3) 3*line(35,3)]  Inductances=[line(35,4) 3*line(35,4)]  Capacitances=[line(35,5) line(35,5)/3]
  36-1 : spsThreePhasePISectionLineLib/Three-Phase PI Section Line  LConnTagsString=a|b|c  RConnTagsString=A|B|C  Length=1  Frequency=60  Resistances=[line(36,3) 3*line(36,3)]  Inductances=[line(36,4) 3*line(36,4)]  Capacitances=[line(36,5) line(36,5)/3]
  47 : spsThreePhaseVIMeasurementLib/Three-Phase V-I Measurement  VoltageMeasurement=phase-to-phase  SetLabelV=on  LabelV=Vabc_47  Vpu=off  VpuLL=on  CurrentMeasurement=no  SetLabelI=off  LabelI=Iabc  Ipu=off  Pbase=100e6  Vbase=Bus(47,2)*1e3  OutputType=Complex  PhasorSimulation=off  PSBequivalent=0
  53 : spsThreePhaseVIMeasurementLib/Three-Phase V-I Measurement  VoltageMeasurement=phase-to-phase  SetLabelV=on  LabelV=Vabc_53  Vpu=off  VpuLL=on  CurrentMeasurement=no  SetLabelI=off  LabelI=Iabc  Ipu=off  Pbase=100e6  Vbase=Bus(53,2)*1e3  OutputType=Complex  PhasorSimulation=off  PSBequivalent=0
  54 : spsThreePhaseVIMeasurementLib/Three-Phase V-I Measurement  VoltageMeasurement=phase-to-phase  SetLabelV=on  LabelV=Vabc_54  Vpu=off  VpuLL=on  CurrentMeasurement=no  SetLabelI=off  LabelI=Iabc  Ipu=off  Pbase=100e6  Vbase=Bus(54,2)*1e3  OutputType=Complex  PhasorSimulation=off  PSBequivalent=0
  63-1 : spsThreePhasePISectionLineLib/Three-Phase PI Section Line  LConnTagsString=a|b|c  RConnTagsString=A|B|C  Length=1  Frequency=60  Resistances=[line(63,3) 3*line(63,3)]  Inductances=[line(63,4) 3*line(63,4)]  Capacitances=[line(63,5) line(63,5)/3]
  66-1 : spsThreePhasePISectionLineLib/Three-Phase PI Section Line  LConnTagsString=a|b|c  RConnTagsString=A|B|C  Length=1  Frequency=60  Resistances=[line(66,3) 3*line(66,3)]  Inductances=[line(66,4) 3*line(66,4)]  Capacitances=[line(66,5) line(66,5)/3]
  G1 : Subsystem
  G8 : Subsystem
  G9 : Subsystem
  Load Flow Bus : spsLoadFlowBusLib/Load Flow Bus  LConnTagsString=a  Phases=single  Connectors=on one side  ID=BUS_01  Vbase=13.8e3  Vref=1.045  Vangle=0  VLF=1.045  VLFb=1  VLFc=1  angleLF=-3.223  angleLFb=0  angleLFc=0
  Load Flow Bus1 : spsLoadFlowBusLib/Load Flow Bus  LConnTagsString=a  Phases=single  Connectors=on one side  ID=BUS_09  Vbase=13.8e3  Vref=1.025  Vangle=0  VLF=1.025  VLFb=1  VLFc=1  angleLF=3.208  angleLFb=0  angleLFc=0
  Load Flow Bus10 : spsLoadFlowBusLib/Load Flow Bus  LConnTagsString=a  Phases=single  Connectors=on one side  ID=BUS_54  Vbase=138e3  Vref=1  Vangle=0  VLF=1.016  VLFb=1  VLFc=1  angleLF=24.39  angleLFb=0  angleLFc=0
  Load Flow Bus2 : spsLoadFlowBusLib/Load Flow Bus  LConnTagsString=a  Phases=single  Connectors=on one side  ID=BUS_26  Vbase=138e3  Vref=1  Vangle=0  VLF=1.035  VLFb=1  VLFc=1  angleLF=25.02  angleLFb=0  angleLFc=0
  Load Flow Bus3 : spsLoadFlowBusLib/Load Flow Bus  LConnTagsString=a  Phases=single  Connectors=on one side  ID=BUS_27  Vbase=138e3  Vref=1  Vangle=0  VLF=1.025  VLFb=1  VLFc=1  angleLF=24.61  angleLFb=0  angleLFc=0
  Load Flow Bus4 : spsLoadFlowBusLib/Load Flow Bus  LConnTagsString=a  Phases=single  Connectors=on one side  ID=BUS_08  Vbase=13.8e3  Vref=1.03  Vangle=0  VLF=1.03  VLFb=1  VLFc=1  angleLF=2.567  angleLFb=0  angleLFc=0
  Load Flow Bus5 : spsLoadFlowBusLib/Load Flow Bus  LConnTagsString=a  Phases=single  Connectors=on one side  ID=BUS_25  Vbase=138e3  Vref=1  Vangle=0  VLF=1.031  VLFb=1  VLFc=1  angleLF=25.81  angleLFb=0  angleLFc=0
  Load Flow Bus6 : spsLoadFlowBusLib/Load Flow Bus  LConnTagsString=a  Phases=single  Connectors=on one side  ID=BUS_28  Vbase=138e3  Vref=1  Vangle=0  VLF=1.028  VLFb=1  VLFc=1  angleLF=25.71  angleLFb=0  angleLFc=0
  Load Flow Bus7 : spsLoadFlowBusLib/Load Flow Bus  LConnTagsString=a  Phases=single  Connectors=on one side  ID=BUS_29  Vbase=138e3  Vref=1  Vangle=0  VLF=1.019  VLFb=1  VLFc=1  angleLF=26.38  angleLFb=0  angleLFc=0
  Load Flow Bus8 : spsLoadFlowBusLib/Load Flow Bus  LConnTagsString=a  Phases=single  Connectors=on one side  ID=BUS_47  Vbase=138e3  Vref=1  Vangle=0  VLF=1.013  VLFb=1  VLFc=1  angleLF=17.53  angleLFb=0  angleLFc=0
  Load Flow Bus9 : spsLoadFlowBusLib/Load Flow Bus  LConnTagsString=a  Phases=single  Connectors=on one side  ID=BUS_53  Vbase=138e3  Vref=1  Vangle=0  VLF=1.006  VLFb=1  VLFc=1  angleLF=18.11  angleLFb=0  angleLFc=0
  Snubber 5 : spsThreePhaseSeriesRLCLoadLib/Three-Phase Series RLC Load  LConnTagsString=A|B|C  Configuration=Y (grounded)  NominalVoltage=13.8e3  Vabc=[1e3 1e3 1e3]  Vabcp=[1e3 1e3 1e3]  NominalFrequency=60  UnbalancedPower=off  ActivePower=1000000  InductivePower=0  CapacitivePower=10000000  Pabc=[10e3 9e3 11e3]  QLabc=[100 90 110]  QCabc=[100 90 110]  Pabcp=[10e3 9e3 11e3]  QLabcp=[100 90 110]  QCabcp=[100 90 110]  Measurements=None  LoadType=constant Z
  Snubber 6 : spsThreePhaseSeriesRLCLoadLib/Three-Phase Series RLC Load  LConnTagsString=A|B|C  Configuration=Y (grounded)  NominalVoltage=13.8e3  Vabc=[1e3 1e3 1e3]  Vabcp=[1e3 1e3 1e3]  NominalFrequency=60  UnbalancedPower=off  ActivePower=1000000  InductivePower=0  CapacitivePower=10000000  Pabc=[10e3 9e3 11e3]  QLabc=[100 90 110]  QCabc=[100 90 110]  Pabcp=[10e3 9e3 11e3]  QLabcp=[100 90 110]  QCabcp=[100 90 110]  Measurements=None  LoadType=constant Z
  Snubber 7 : spsThreePhaseSeriesRLCLoadLib/Three-Phase Series RLC Load  LConnTagsString=A|B|C  Configuration=Y (grounded)  NominalVoltage=13.8e3  Vabc=[1e3 1e3 1e3]  Vabcp=[1e3 1e3 1e3]  NominalFrequency=60  UnbalancedPower=off  ActivePower=1000000  InductivePower=0  CapacitivePower=10000000  Pabc=[10e3 9e3 11e3]  QLabc=[100 90 110]  QCabc=[100 90 110]  Pabcp=[10e3 9e3 11e3]  QLabcp=[100 90 110]  QCabcp=[100 90 110]  Measurements=None  LoadType=constant Z
  T01-54 : spsThreePhaseTransformerTwoWindingsLib/Three-Phase Transformer (Two Windings)  Winding1Connection=Delta (D1)  Winding2Connection=Yg  CoreType=Three single-phase transformers  SetSaturation=off  Hysteresis=off  DataFile='hysteresis'  SetInitialFlux=off  Measurements=None  UNITS=pu  NominalPower=[ 100e6 , 60 ]  Winding1=[ 13.8e3 , 0.0002 , 0 ]  Winding2=[ 138e3 , 0.0002, 0.0181]  Rm=500  Lm=500  L0=0.5  Saturation=[ 0,0 ; 0.0024,1.2 ; 1.0,1.52 ]  InitialFluxes=[ 0.8 , -0.8 , 0.7 ]  BreakLoop=off  DiscreteSolver=Trapezoidal robust  DataType=off  TransfoNumber=1
  T08-25 : spsThreePhaseTransformerTwoWindingsLib/Three-Phase Transformer (Two Windings)  Winding1Connection=Delta (D1)  Winding2Connection=Yg  CoreType=Three single-phase transformers  SetSaturation=off  Hysteresis=off  DataFile='hysteresis'  SetInitialFlux=off  Measurements=None  UNITS=pu  NominalPower=[ 100e6 , 60 ]  Winding1=[ 13.8e3 , 0.0003 , 0 ]  Winding2=[ 138e3 , 0.0003, 0.0232]  Rm=500  Lm=500  L0=0.5  Saturation=[ 0,0 ; 0.0024,1.2 ; 1.0,1.52 ]  InitialFluxes=[ 0.8 , -0.8 , 0.7 ]  BreakLoop=off  DiscreteSolver=Trapezoidal robust  DataType=off  TransfoNumber=1
  T09-29 : spsThreePhaseTransformerTwoWindingsLib/Three-Phase Transformer (Two Windings)  Winding1Connection=Delta (D1)  Winding2Connection=Yg  CoreType=Three single-phase transformers  SetSaturation=off  Hysteresis=off  DataFile='hysteresis'  SetInitialFlux=off  Measurements=None  UNITS=pu  NominalPower=[ 100e6 , 60 ]  Winding1=[ 13.8e3 , 0.0004 , 0 ]  Winding2=[ 138e3 , 0.0004 , 0.0156]  Rm=500  Lm=500  L0=0.5  Saturation=[ 0,0 ; 0.0024,1.2 ; 1.0,1.52 ]  InitialFluxes=[ 0.8 , -0.8 , 0.7 ]  BreakLoop=off  DiscreteSolver=Trapezoidal robust  DataType=off  TransfoNumber=1
  load25 : spsThreePhaseParallelRLCLoadLib/Three-Phase Parallel RLC Load  LConnTagsString=A|B|C  Configuration=Y (grounded)  NominalVoltage=(138000)*1.03069  Vabc=[1e3 1e3 1e3]  Vabcp=[1e3 1e3 1e3]  NominalFrequency=60  UnbalancedPower=off  ActivePower=224000000  InductivePower=47000000  CapacitivePower=0  Pabc=[10e3 9e3 11e3]  QLabc=[100 90 110]  QCabc=[100 90 110]  Pabcp=[10e3 9e3 11e3]  QLabcp=[100 90 110]  QCabcp=[100 90 110]  Measurements=None  LoadType=constant PQ
  load26 : spsThreePhaseParallelRLCLoadLib/Three-Phase Parallel RLC Load  LConnTagsString=A|B|C  Configuration=Y (grounded)  NominalVoltage=(138000)*1.03482  Vabc=[1e3 1e3 1e3]  Vabcp=[1e3 1e3 1e3]  NominalFrequency=60  UnbalancedPower=off  ActivePower=50000000  InductivePower=7000000  CapacitivePower=0  Pabc=[10e3 9e3 11e3]  QLabc=[100 90 110]  QCabc=[100 90 110]  Pabcp=[10e3 9e3 11e3]  QLabcp=[100 90 110]  QCabcp=[100 90 110]  Measurements=None  LoadType=constant PQ
  load27 : spsThreePhaseParallelRLCLoadLib/Three-Phase Parallel RLC Load  LConnTagsString=A|B|C  Configuration=Y (grounded)  NominalVoltage=(138000)*1.02463  Vabc=[1e3 1e3 1e3]  Vabcp=[1e3 1e3 1e3]  NominalFrequency=60  UnbalancedPower=off  ActivePower=130000000  InductivePower=20000000  CapacitivePower=0  Pabc=[10e3 9e3 11e3]  QLabc=[100 90 110]  QCabc=[100 90 110]  Pabcp=[10e3 9e3 11e3]  QLabcp=[100 90 110]  QCabcp=[100 90 110]  Measurements=None  LoadType=constant PQ
  load28 : spsThreePhaseParallelRLCLoadLib/Three-Phase Parallel RLC Load  LConnTagsString=A|B|C  Configuration=Y (grounded)  NominalVoltage=(138000)*1.0279  Vabc=[1e3 1e3 1e3]  Vabcp=[1e3 1e3 1e3]  NominalFrequency=60  UnbalancedPower=off  ActivePower=50000000  InductivePower=7000000  CapacitivePower=0  Pabc=[10e3 9e3 11e3]  QLabc=[100 90 110]  QCabc=[100 90 110]  Pabcp=[10e3 9e3 11e3]  QLabcp=[100 90 110]  QCabcp=[100 90 110]  Measurements=None  LoadType=constant PQ
  load29 : spsThreePhaseParallelRLCLoadLib/Three-Phase Parallel RLC Load  LConnTagsString=A|B|C  Configuration=Y (grounded)  NominalVoltage=(138000)*1.01949  Vabc=[1e3 1e3 1e3]  Vabcp=[1e3 1e3 1e3]  NominalFrequency=60  UnbalancedPower=off  ActivePower=680000000  InductivePower=106000000  CapacitivePower=0  Pabc=[10e3 9e3 11e3]  QLabc=[100 90 110]  QCabc=[100 90 110]  Pabcp=[10e3 9e3 11e3]  QLabcp=[100 90 110]  QCabcp=[100 90 110]  Measurements=None  LoadType=constant PQ
  load47 : spsThreePhaseParallelRLCLoadLib/Three-Phase Parallel RLC Load  LConnTagsString=A|B|C  Configuration=Y (grounded)  NominalVoltage=(138000)*1.01263  Vabc=[1e3 1e3 1e3]  Vabcp=[1e3 1e3 1e3]  NominalFrequency=60  UnbalancedPower=off  ActivePower=203000000  InductivePower=33000000  CapacitivePower=0  Pabc=[10e3 9e3 11e3]  QLabc=[100 90 110]  QCabc=[100 90 110]  Pabcp=[10e3 9e3 11e3]  QLabcp=[100 90 110]  QCabcp=[100 90 110]  Measurements=None  LoadType=constant PQ
  load53 : spsThreePhaseParallelRLCLoadLib/Three-Phase Parallel RLC Load  LConnTagsString=A|B|C  Configuration=Y (grounded)  NominalVoltage=(138000)*1.00612  Vabc=[1e3 1e3 1e3]  Vabcp=[1e3 1e3 1e3]  NominalFrequency=60  UnbalancedPower=off  ActivePower=253000000  InductivePower=119000000  CapacitivePower=0  Pabc=[10e3 9e3 11e3]  QLabc=[100 90 110]  QCabc=[100 90 110]  Pabcp=[10e3 9e3 11e3]  QLabcp=[100 90 110]  QCabcp=[100 90 110]  Measurements=None  LoadType=constant PQ
  a27 : PMIOPort  Tag=PMCPort  Side=Right
  b27 : PMIOPort  Tag=PMCPort  Port=2  Side=Right
  c27 : PMIOPort  Tag=PMCPort  Port=3  Side=Right
  A54 : PMIOPort  Tag=PMCPort  Port=4  Side=Right
  B54 : PMIOPort  Tag=PMCPort  Port=5  Side=Right
  C54 : PMIOPort  Tag=PMCPort  Port=6  Side=Right
  a53 : PMIOPort  Tag=PMCPort  Port=7  Side=Right
  b53 : PMIOPort  Tag=PMCPort  Port=8  Side=Right
  c53 : PMIOPort  Tag=PMCPort  Port=9  Side=Right
  a47 : PMIOPort  Tag=PMCPort  Port=10  Side=Right
  b47 : PMIOPort  Tag=PMCPort  Port=11  Side=Right
  c47 : PMIOPort  Tag=PMCPort  Port=12  Side=Right
  C53 : PMIOPort  Tag=PMCPort  Port=13  Side=Right
  B53 : PMIOPort  Tag=PMCPort  Port=14  Side=Right
  A53 : PMIOPort  Tag=PMCPort  Port=15  Side=Right
  connections:
  T09-29/LConn1 -- Snubber 5/LConn1 -- 09/LConn1 -- Load Flow Bus1/LConn1
  G9/LConn1 -- 09/RConn1
  G9/LConn2 -- 09/RConn2
  G9/LConn3 -- 09/RConn3
  T09-29/LConn3 -- Snubber 5/LConn3 -- 09/LConn3
  T09-29/LConn2 -- Snubber 5/LConn2 -- 09/LConn2
  29/RConn1 -- T09-29/RConn1
  29/RConn2 -- T09-29/RConn2
  29/RConn3 -- T09-29/RConn3
  33-1/RConn1 -- load29/LConn1 -- 29/LConn1 -- Load Flow Bus7/LConn1 -- 36-1/RConn1
  36-1/RConn2 -- load29/LConn2 -- 29/LConn2 -- 33-1/RConn2
  36-1/RConn3 -- load29/LConn3 -- 29/LConn3 -- 33-1/RConn3
  36-1/LConn1 -- 28/RConn1
  36-1/LConn2 -- 28/RConn2
  36-1/LConn3 -- 28/RConn3
  32-1/RConn1 -- load28/LConn1 -- Load Flow Bus6/LConn1 -- 28/LConn1
  32-1/RConn2 -- load28/LConn2 -- 28/LConn2
  32-1/RConn3 -- load28/LConn3 -- 28/LConn3
  32-1/LConn1 -- 33-1/LConn1 -- 26/RConn1 -- 29-1/LConn1
  32-1/LConn2 -- 33-1/LConn2 -- 26/RConn2 -- 29-1/LConn2
  26/RConn3 -- 32-1/LConn3 -- 33-1/LConn3 -- 29-1/LConn3
  load27/LConn1 -- 35-1/RConn1 -- Load Flow Bus3/LConn1 -- 27/LConn1
  load27/LConn2 -- 27/LConn2 -- 35-1/RConn2
  load27/LConn3 -- 27/LConn3 -- 35-1/RConn3
  T08-25/RConn1 -- 25/RConn1
  T08-25/RConn2 -- 25/RConn2
  T08-25/RConn3 -- 25/RConn3
  load26/LConn1 -- 31-1/RConn1 -- Load Flow Bus2/LConn1 -- 26/LConn1
  load26/LConn2 -- 31-1/RConn2 -- 26/LConn2
  load26/LConn3 -- 31-1/RConn3 -- 26/LConn3
  G8/LConn1 -- 08/RConn1
  G8/LConn2 -- 08/RConn2
  G8/LConn3 -- 08/RConn3
  T08-25/LConn1 -- Load Flow Bus4/LConn1 -- Snubber 6/LConn1 -- 08/LConn1
  T08-25/LConn2 -- Snubber 6/LConn2 -- 08/LConn2
  T08-25/LConn3 -- Snubber 6/LConn3 -- 08/LConn3
  25/LConn1 -- Load Flow Bus5/LConn1 -- 30-1/RConn1 -- load25/LConn1 -- 29-1/RConn1
  25/LConn2 -- 30-1/RConn2 -- load25/LConn2 -- 29-1/RConn2
  25/LConn3 -- 30-1/RConn3 -- load25/LConn3 -- 29-1/RConn3
  30-1/LConn1 -- T01-54/RConn1 -- 54/RConn1
  30-1/LConn2 -- T01-54/RConn2 -- 54/RConn2
  30-1/LConn3 -- T01-54/RConn3 -- 54/RConn3
  T01-54/LConn1 -- 01/LConn1 -- Snubber 7/LConn1 -- Load Flow Bus/LConn1
  T01-54/LConn2 -- 01/LConn2 -- Snubber 7/LConn2
  T01-54/LConn3 -- 01/LConn3 -- Snubber 7/LConn3
  G1/LConn1 -- 01/RConn1
  G1/LConn2 -- 01/RConn2
  G1/LConn3 -- 01/RConn3
  66-1/RConn1 -- Load Flow Bus10/LConn1 -- 54/LConn1 -- A54/RConn1
  66-1/RConn2 -- 54/LConn2 -- B54/RConn1
  66-1/RConn3 -- C54/RConn1 -- 54/LConn3
  a53/RConn1 -- 53/RConn1 -- 66-1/LConn1 -- 35-1/LConn1
  b53/RConn1 -- 53/RConn2 -- 66-1/LConn2 -- 35-1/LConn2
  c53/RConn1 -- 53/RConn3 -- 66-1/LConn3 -- 35-1/LConn3
  63-1/RConn1 -- load53/LConn1 -- Load Flow Bus9/LConn1 -- 53/LConn1 -- A53/RConn1
  53/LConn2 -- load53/LConn2 -- 63-1/RConn2 -- B53/RConn1
  63-1/RConn3 -- 53/LConn3 -- load53/LConn3 -- C53/RConn1
  47/RConn1 -- 63-1/LConn1 -- a47/RConn1
  47/RConn2 -- 63-1/LConn2 -- b47/RConn1
  47/RConn3 -- 63-1/LConn3 -- c47/RConn1
  31-1/LConn1 -- a27/RConn1 -- 27/RConn1
  27/RConn2 -- b27/RConn1 -- 31-1/LConn2
  27/RConn3 -- c27/RConn1 -- 31-1/LConn3
  load47/LConn1 -- Load Flow Bus8/LConn1 -- 47/LConn1
  load47/LConn2 -- 47/LConn2
  load47/LConn3 -- 47/LConn3
